simulink model "drone_dyn"  (R2026a)
settings: Solver=VariableStepAuto  StopTime=20
values from neighbouring files (symbols this model uses):
  drone =     [params.mat]
libraries: matrix_library x1
settings Model: Creator=flow  LastModifiedBy=flow

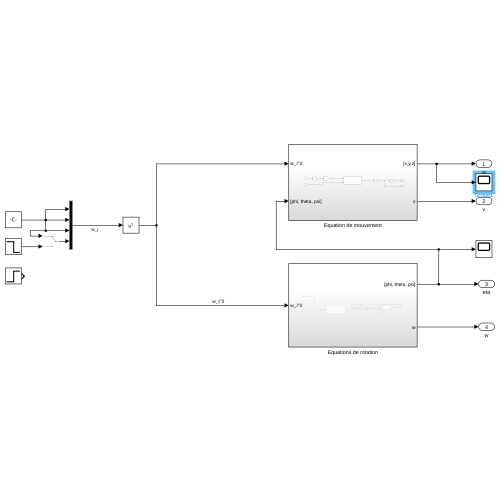
[thumbnail: Simulink's stored preview of the top-level diagram]
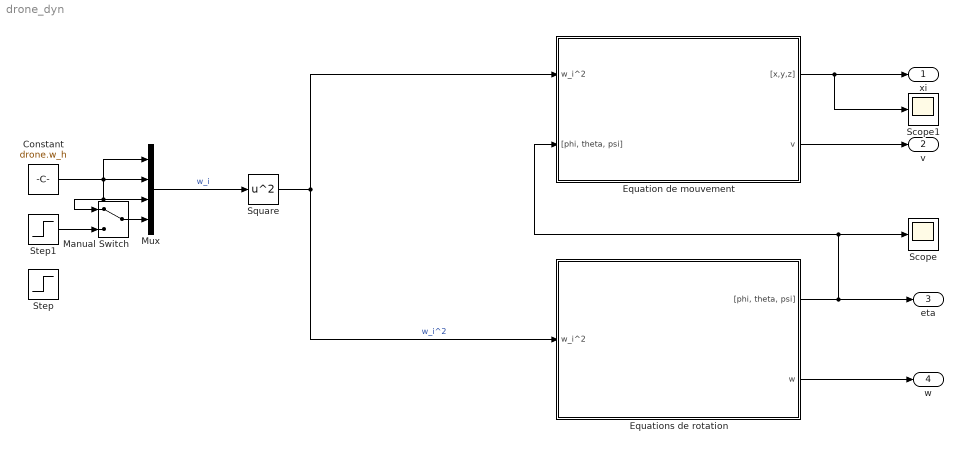
== system drone_dyn ==
  Constant : Constant  Value=drone.w_h
  Equation de mouvement : Subsystem
  Equations de rotation : Subsystem
  Manual Switch : ManualSwitch
  Mux : Mux
  Scope : Scope
      settings: ActiveDisplayYMinimum=-1  ActiveDisplayYMaximum=1
  Scope1 : Scope
      settings: ActiveDisplayYMinimum=-3.0020430585864228E-15  ActiveDisplayYMaximum=2.7018387527277811E-14
  Square : Math  Operator=square
  Step : Step  Time=10  InitialValue=drone.w_h  FinalValue=drone.w_h*1.2  SampleTime=0
  Step1 : Step  Time=10  InitialValue=drone.w_h  FinalValue=drone.w_h*0.1  SampleTime=0
  xi : Outport
  v : Outport  Port=2
  eta : Outport  Port=3
  w : Outport  Port=4
  wires:
  Constant/1 -> Mux/1, Mux/3, Manual Switch/1, Mux/2
  Mux/1 -> Square/1  "w_i"
  Square/1 -> Equations de rotation/1(w_i^2), Equation de mouvement/1(w_i^2)  "w_i^2"
  Step1/1 -> Manual Switch/2
  Manual Switch/1 -> Mux/4
  Equation de mouvement/1("[x,y,z]") -> Scope1/1, xi/1
  Equations de rotation/1("[phi, theta, psi]") -> Equation de mouvement/2("[phi, theta, psi]"), Scope/1, eta/1
  Equation de mouvement/2(v) -> v/1
  Equations de rotation/2(w) -> w/1

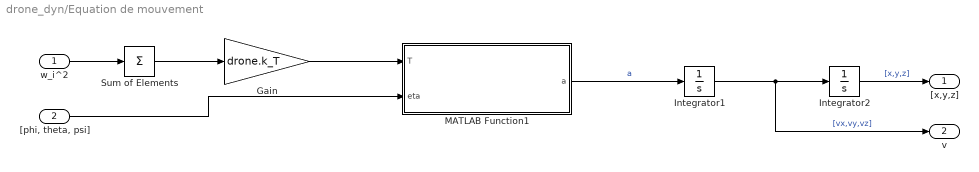
== system drone_dyn/Equation de mouvement ==
  w_i^2 : Inport
  "[phi, theta, psi]" : Inport  Port=2
  Gain : Gain  Gain=drone.k_T
  Integrator1 : Integrator
  Integrator2 : Integrator
  MATLAB Function1 : MATLAB Function  TreatAsAtomicUnit=on
  Sum of Elements : Sum  Inputs=+
  "[x,y,z]" : Outport
  v : Outport  Port=2
  wires:
  MATLAB Function1/1(a) -> Integrator1/1  "a"
  Integrator1/1 -> v/1, Integrator2/1  "[vx,vy,vz]"
  Gain/1 -> MATLAB Function1/1(T)
  Sum of Elements/1 -> Gain/1
  Integrator2/1 -> "[x,y,z]"/1  "[x,y,z]"
  w_i^2/1 -> Sum of Elements/1
  "[phi, theta, psi]"/1 -> MATLAB Function1/2(eta)

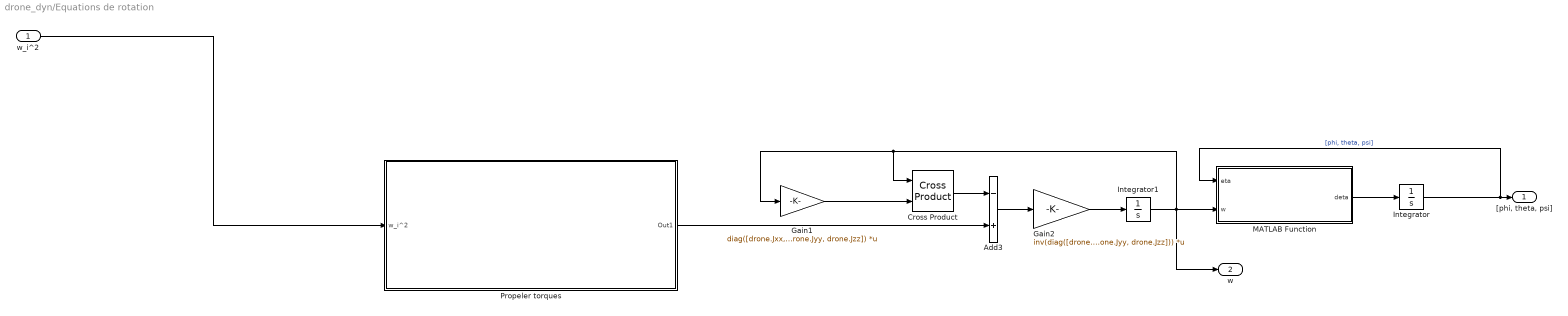
== system drone_dyn/Equations de rotation ==
  w_i^2 : Inport
  Add3 : Sum  Inputs=-+
  Cross Product : matrix_library/Cross Product
  Gain1 : Gain  Gain=diag([drone.Jxx, drone.Jyy, drone.Jzz])  Multiplication=Matrix(K*u) (u vector)
  Gain2 : Gain  Gain=inv(diag([drone.Jxx, drone.Jyy, drone.Jzz]))  Multiplication=Matrix(K*u) (u vector)
  Integrator : Integrator
  Integrator1 : Integrator
  MATLAB Function : MATLAB Function  TreatAsAtomicUnit=on
  Propeler torques : Subsystem
  "[phi, theta, psi]" : Outport
  w : Outport  Port=2
  wires:
  MATLAB Function/1(deta) -> Integrator/1
  Add3/1 -> Gain2/1
  w_i^2/1 -> Propeler torques/1(w_i^2)
  Gain1/1 -> Cross Product/2
  Cross Product/1 -> Add3/1
  Propeler torques/1(Out1) -> Add3/2
  Integrator/1 -> MATLAB Function/1(eta), "[phi, theta, psi]"/1  "[phi, theta, psi]"
  Gain2/1 -> Integrator1/1
  Integrator1/1 -> w/1, Gain1/1, Cross Product/1, MATLAB Function/2(w)

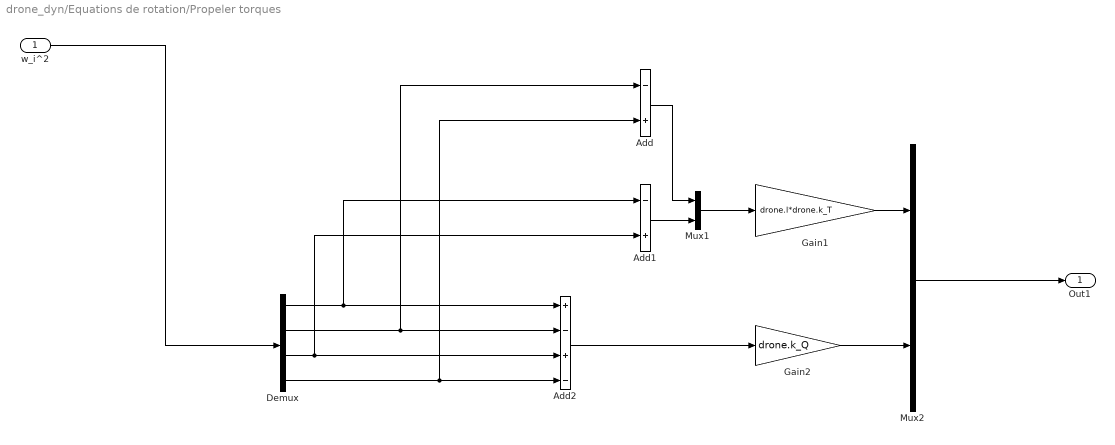
== system drone_dyn/Equations de rotation/Propeler torques ==
  w_i^2 : Inport
  Add : Sum  Inputs=-+
  Add1 : Sum  Inputs=-+
  Add2 : Sum  Inputs=+-+-
  Demux : Demux
  Gain1 : Gain  Gain=drone.l*drone.k_T
  Gain2 : Gain  Gain=drone.k_Q
  Mux1 : Mux  Inputs=2
  Mux2 : Mux  Inputs=2
  Out1 : Outport
  wires:
  Add1/1 -> Mux1/2
  Demux/3 -> Add2/3, Add1/2
  Gain2/1 -> Mux2/2
  Mux1/1 -> Gain1/1
  Demux/4 -> Add2/4, Add/2
  Gain1/1 -> Mux2/1
  w_i^2/1 -> Demux/1
  Demux/1 -> Add2/1, Add1/1
  Mux2/1 -> Out1/1
  Add2/1 -> Gain2/1
  Demux/2 -> Add2/2, Add/1
  Add/1 -> Mux1/1

== matlab function drone_dyn/Equations de rotation/MATLAB Function ==
  data: eta input size=[3 1]; deta output size=[3 1]; w input size=[3 1]
function deta = fcn(eta,w)

phi = eta(1);
theta = eta(2);
psi = eta(3);

cphi    = cos(phi);
sphi    = sin(phi);
ctheta  = cos(theta);
stheta  = sin(theta);
ttheta  = stheta/ctheta;
cpsi    = cos(psi);
spsi    = sin(psi);



% Matrice de dérivation des angles d'euler
W = [1  sphi*ttheta cphi*ttheta;
    0  cphi        -sphi;
    0  sphi/ctheta cphi/ctheta];

% eta = [phi; theta; psi]
deta = W*w;

== matlab function drone_dyn/Equation de mouvement/MATLAB Function1 ==
  data: T input size=1; a output size=[3 1]; eta input size=[3 1]
function a = fcn(T, eta)

m = 0.5;
g = 9.81;

phi = eta(1);
theta = eta(2);
psi = eta(3);

cphi    = cos(phi);
sphi    = sin(phi);
ctheta  = cos(theta);
stheta  = sin(theta);
cpsi    = cos(psi);
spsi    = sin(psi);

% Matrice de transition du repère du quadroptere dans le repere
% terrestre
R = [cpsi*ctheta,  cpsi*stheta*sphi - spsi*cphi,  cpsi*stheta*cphi + spsi*sphi;
    spsi*ctheta,  spsi*stheta*sphi + cpsi*cphi,  spsi*stheta*cphi - cpsi*sphi;
    -stheta,      ctheta*sphi,                   ctheta*cphi];

a = (1/m)*(R*[0;0;T]-[0;0;m*g]);
